simulink model "ZT_VehCtrl_18B_CAN"  (R2018b)
settings: Solver=FixedStepAuto  StartTime=0.0  StopTime=inf  FixedStep=0.005  RelTol=1e-3
InitFcn:
  | mbd_mpc_consistency_checks(bdroot(gcs));
values from neighbouring files (symbols this model uses):
  BatoverTempTh = single(80)    [VCU_INIT.m]
  BRS_PwrValid = single(5)    [VCU_INIT.m]
  BRSEnSpdTh1 = single(10)    [VCU_INIT.m]
  BRSEnSpdTh2 = single(20)    [VCU_INIT.m]
  MCUTempAlarmTh = single (60)    [VCU_INIT.m]
  mps2kmh = single(3.6)    [VCU_INIT.m]
  MtrPwrFac = single(1/9550)    [VCU_INIT.m]
  MtrTempAlarmTh = single (50)    [VCU_INIT.m]
  Padle1Signal1_Th = [PadleSignal1_min,PadleSignal1_max]    [VCU_INIT.m]
  Padle1Signal2_Th = [PadleSignal2_min,PadleSignal2_max]    [VCU_INIT.m]
  PadleSignal1_max = 3.84    [VCU_INIT.m]
  PadleSignal1_min = 0.75    [VCU_INIT.m]
  PadleSignal2_max = 1.92    [VCU_INIT.m]
  PadleSignal2_min = 0.375    [VCU_INIT.m]
  PadleValid = 0.05    [VCU_INIT.m]
  PwrLimFactor = single(0.5)    [VCU_INIT.m]
  Ratio = single(1)    [VCU_INIT.m]
  rpm2mps = single(2*pi/60 * WhlRadius/Ratio)    [VCU_INIT.m]
  SOCLowTh = single(20)    [VCU_INIT.m]
  VehPwrBackwardMax = VehPwrMax * single(0.3)    [VCU_INIT.m]
  VehPwrMax = single(MtrPwrMax * 4)    [VCU_INIT.m]
  VehTrqBackwardMax = VehTrqMax * single(0.3)    [VCU_INIT.m]
  VehTrqMax = single(MtrTrqMax * Ratio *4)    [VCU_INIT.m]
  WhlRadius = single(1)    [VCU_INIT.m]
undefined symbols (not defined in the file or in its folder): Delay_Charge, Delay_Discharge, fifo_0_vect, fifo_1_vect, LQFP, pts1_fifo_0_vect, pts1_fifo_1_vect, pts2_fifo_0_vect, pts2_fifo_1_vect, pts3_fifo_0_vect, pts3_fifo_1_vect, pts4_fifo_0_vect, pts4_fifo_1_vect
libraries: mbd_mpc574x_ec_toolbox x157, canmsglib x74, simulink x38
(part 7 of 12)

== system ZT_VehCtrl_18B_CAN/SigIn/CAN0 / BMS Power Control/UNPACK ==
  ID : Inport
  data : Inport  Port=2
  length : Inport  Port=3
  timestamp : Inport  Port=4
  Action Port : ActionPort
  Bus Creator : BusCreator  Inputs=7  OutDataTypeStr=Bus: CAN_MESSAGE_BUS  NonVirtualBus=on
  Bus Creator1 : BusCreator  Inputs=4
  CAN Unpack6 : canmsglib/CAN Unpack  CANdbFile=D:\VCU\VCU_SL_ZhengZhou\ZT2\模型与接口\CAN_DBC\整车CANA_GBK.dbc  MsgList=(none)  MsgName=BMS_Power_Control  MsgIDType=Standard (11-bit identifier)  MsgIdentifier=499  MsgLength=8  SignalInfo=Power_ChargeContinue$56$16$2$2$1$0$1.000000e-01$0$0$1000$#Power_ChargePeak$40$16$2$2$1$0$1.000000e-01$0$0$1000$#Power_DischargeContinue$24$16$2$2$1$0$1.000000e-01$0$0$1000$#Power_DischargePeak$8$16$2$2$1$0$1.000000e-01$0$0$1000$#  NSignals=4  IDPort=off  TimestampPort=off  ErrorPort=off  RemotePort=off  LengthPort=off  StatusPort=off  StartBits=str2num('[int32(56);int32(40);int32(24);int32(8)]')  SignalSizes=str2num('[int32(16);int32(16);int32(16);int32(16)]')  ByteOrders=str2num('[int32(2);int32(2);int32(2);int32(2)]')  DataTypes=str2num('[int32(2);int32(2);int32(2);int32(2)]')  MultiplexTypes=str2num('[int32(1);int32(1);int32(1);int32(1)]')  MultiplexValues=str2num('[double(0);double(0);double(0);double(0)]')  Factors=str2num('[double(1.000000e-01);double(1.000000e-01);double(1.000000e-01);double(1.000000e-01)]')  Offsets=str2num('[double(0);double(0);double(0);double(0)]')  Minimums=str2num('[double(0);double(0);double(0);double(0)]')  Maximums=str2num('[double(1000);double(1000);double(1000);double(1000)]')  ApplyMinMax=off
      settings: SourceProductName=Simulink Real-Time  SourceProductBaseCode=XP  DataFormat=CANdb specified signals
  Constant1 : Constant  Value=0  OutDataTypeStr=uint8
  Constant4 : Constant  Value=0  OutDataTypeStr=uint8
  Constant5 : Constant  Value=0  OutDataTypeStr=uint8
  Data Type Conversion{,14..15,17} (4 alike) : DataTypeConversion  OutDataTypeStr=uint8
  Data Type Conversion18 : DataTypeConversion  OutDataTypeStr=uint32
  Data Type Conversion19 : DataTypeConversion  OutDataTypeStr=double
  Message : Outport
  wires:
  Constant4/1 -> Data Type Conversion15/1
  length/1 -> Data Type Conversion14/1
  data/1 -> Bus Creator/7  "Data"
  Data Type Conversion18/1 -> Bus Creator/5  "ID"
  Constant1/1 -> Data Type Conversion/1
  Constant5/1 -> Data Type Conversion17/1
  ID/1 -> Data Type Conversion18/1
  Data Type Conversion19/1 -> Bus Creator/6  "Timestamp"
  timestamp/1 -> Data Type Conversion19/1
  Data Type Conversion17/1 -> Bus Creator/4  "Error"
  Bus Creator/1 -> CAN Unpack6/1  "CAN_Msg_In"
  Data Type Conversion/1 -> Bus Creator/1  "Extended"
  Data Type Conversion14/1 -> Bus Creator/2  "Length"
  Data Type Conversion15/1 -> Bus Creator/3  "Remote"
  Bus Creator1/1 -> Message/1

== system ZT_VehCtrl_18B_CAN/SigIn/CAN0 /ACU1/UNPACK ==
  ID : Inport
  data : Inport  Port=2
  length : Inport  Port=3
  timestamp : Inport  Port=4
  Action Port : ActionPort  ActionType=case
  Add : Sum
  Bus Creator : BusCreator  Inputs=7  OutDataTypeStr=Bus: CAN_MESSAGE_BUS  NonVirtualBus=on
  Bus Creator1 : BusCreator  Inputs=5
  CAN Unpack6 : canmsglib/CAN Unpack  CANdbFile=D:\VCU\VCU_SL_ZhengZhou\ZT2\模型与接口\CAN_DBC\动力CANB_GBK.dbc  MsgList=(none)  MsgName=ACU1  MsgIDType=Extended (29-bit identifier)  MsgIdentifier=201893786  MsgLength=8  SignalInfo=FaultCode$56$8$1$2$1$0$1$0$0$255$#InputVoltage$32$16$1$1$1$0$1.000000e-01$-1000$-1000$1000$#OutputCurrent$16$16$1$1$1$0$1.000000e-01$-1000$-1000$1000$#OutputVoltage$0$16$1$1$1$0$1.000000e-01$-1000$-1000$1000$#Temp$48$8$1$1$1$0$1$-50$-50$200$#  NSignals=5  IDPort=off  TimestampPort=off  ErrorPort=off  RemotePort=off  LengthPort=off  StatusPort=off  StartBits=str2num('[int32(56);int32(32);int32(16);int32(0);int32(48)]')  SignalSizes=str2num('[int32(8);int32(16);int32(16);int32(16);int32(8)]')  ByteOrders=str2num('[int32(1);int32(1);int32(1);int32(1);int32(1)]')  DataTypes=str2num('[int32(2);int32(1);int32(1);int32(1);int32(1)]')  MultiplexTypes=str2num('[int32(1);int32(1);int32(1);int32(1);int32(1)]')  MultiplexValues=str2num('[double(0);double(0);double(0);double(0);double(0)]')  Factors=str2num('[double(1);double(1.000000e-01);double(1.000000e-01);double(1.000000e-01);double(1)]')  Offsets=str2num('[double(0);double(-1000);double(-1000);double(-1000);double(-50)]')  Minimums=str2num('[double(0);double(-1000);double(-1000);double(-1000);double(-50)]')  Maximums=str2num('[double(255);double(1000);double(1000);double(1000);double(200)]')  ApplyMinMax=off
      settings: SourceProductName=Simulink Real-Time  SourceProductBaseCode=XP  DataFormat=CANdb specified signals
  Constant : Constant  OutDataTypeStr=uint8
  Constant1 : Constant  OutDataTypeStr=uint8
  Constant4 : Constant  Value=0  OutDataTypeStr=uint8
  Constant5 : Constant  Value=0  OutDataTypeStr=uint8
  Data Store Read : DataStoreRead  DataStoreName=Cnt_ACU1
  Data Store Write : DataStoreWrite  DataStoreName=Cnt_ACU1
  Data Type Conversion{,14..15,17} (4 alike) : DataTypeConversion  OutDataTypeStr=uint8
  Data Type Conversion{1..5} (5 alike) : DataTypeConversion  OutDataTypeStr=single
  Data Type Conversion18 : DataTypeConversion  OutDataTypeStr=uint32
  Data Type Conversion19 : DataTypeConversion  OutDataTypeStr=double
  Message : Outport
  wires:
  Constant4/1 -> Data Type Conversion15/1
  length/1 -> Data Type Conversion14/1
  data/1 -> Bus Creator/7  "Data"
  Data Type Conversion18/1 -> Bus Creator/5  "ID"
  Constant1/1 -> Data Type Conversion/1
  Constant5/1 -> Data Type Conversion17/1
  ID/1 -> Data Type Conversion18/1
  Data Type Conversion19/1 -> Bus Creator/6  "Timestamp"
  timestamp/1 -> Data Type Conversion19/1
  Data Type Conversion17/1 -> Bus Creator/4  "Error"
  Bus Creator/1 -> CAN Unpack6/1  "CAN_Msg_In"
  Data Type Conversion/1 -> Bus Creator/1  "Extended"
  Data Type Conversion14/1 -> Bus Creator/2  "Length"
  Data Type Conversion15/1 -> Bus Creator/3  "Remote"
  Bus Creator1/1 -> Message/1
  CAN Unpack6/1 -> Data Type Conversion1/1
  CAN Unpack6/2 -> Data Type Conversion2/1
  CAN Unpack6/3 -> Data Type Conversion3/1
  CAN Unpack6/4 -> Data Type Conversion4/1
  CAN Unpack6/5 -> Data Type Conversion5/1
  Data Type Conversion1/1 -> Bus Creator1/1  "FaultCode"
  Data Type Conversion2/1 -> Bus Creator1/2  "InputVoltage"
  Data Type Conversion3/1 -> Bus Creator1/3  "OutputCurrent"
  Data Type Conversion4/1 -> Bus Creator1/4  "OutputVoltage"
  Data Type Conversion5/1 -> Bus Creator1/5  "Temp"
  Constant/1 -> Add/2
  Data Store Read/1 -> Add/1
  Add/1 -> Data Store Write/1

== system ZT_VehCtrl_18B_CAN/SigIn/CAN0 /ACU2/UNPACK ==
  ID : Inport
  data : Inport  Port=2
  length : Inport  Port=3
  timestamp : Inport  Port=4
  Action Port : ActionPort  ActionType=case
  Add : Sum
  Bus Creator : BusCreator  Inputs=7  OutDataTypeStr=Bus: CAN_MESSAGE_BUS  NonVirtualBus=on
  Bus Creator1 : BusCreator  Inputs=5
  CAN Unpack6 : canmsglib/CAN Unpack  CANdbFile=D:\VCU\VCU_SL_ZhengZhou\ZT2\模型与接口\CAN_DBC\动力CANB_GBK.dbc  MsgList=(none)  MsgName=ACU2  MsgIDType=Extended (29-bit identifier)  MsgIdentifier=201959323  MsgLength=8  SignalInfo=CurrentU$32$16$1$1$1$0$1.000000e-01$-1000$-1000$1000$#CurrentV$16$16$1$1$1$0$1.000000e-01$-1000$-1000$1000$#CurrentW$0$16$1$1$1$0$1.000000e-01$-1000$-1000$1000$#FaultCode$56$8$1$2$1$0$1$0$0$255$#Temp$48$8$1$1$1$0$1$-50$-50$200$#  NSignals=5  IDPort=off  TimestampPort=off  ErrorPort=off  RemotePort=off  LengthPort=off  StatusPort=off  StartBits=str2num('[int32(32);int32(16);int32(0);int32(56);int32(48)]')  SignalSizes=str2num('[int32(16);int32(16);int32(16);int32(8);int32(8)]')  ByteOrders=str2num('[int32(1);int32(1);int32(1);int32(1);int32(1)]')  DataTypes=str2num('[int32(1);int32(1);int32(1);int32(2);int32(1)]')  MultiplexTypes=str2num('[int32(1);int32(1);int32(1);int32(1);int32(1)]')  MultiplexValues=str2num('[double(0);double(0);double(0);double(0);double(0)]')  Factors=str2num('[double(1.000000e-01);double(1.000000e-01);double(1.000000e-01);double(1);double(1)]')  Offsets=str2num('[double(-1000);double(-1000);double(-1000);double(0);double(-50)]')  Minimums=str2num('[double(-1000);double(-1000);double(-1000);double(0);double(-50)]')  Maximums=str2num('[double(1000);double(1000);double(1000);double(255);double(200)]')  ApplyMinMax=off
      settings: SourceProductName=Simulink Real-Time  SourceProductBaseCode=XP  DataFormat=CANdb specified signals
  Constant : Constant  OutDataTypeStr=uint8
  Constant1 : Constant  OutDataTypeStr=uint8
  Constant4 : Constant  Value=0  OutDataTypeStr=uint8
  Constant5 : Constant  Value=0  OutDataTypeStr=uint8
  Data Store Read : DataStoreRead  DataStoreName=Cnt_ACU2
  Data Store Write : DataStoreWrite  DataStoreName=Cnt_ACU2
  Data Type Conversion{,14..15,17} (4 alike) : DataTypeConversion  OutDataTypeStr=uint8
  Data Type Conversion{1..5} (5 alike) : DataTypeConversion  OutDataTypeStr=single
  Data Type Conversion18 : DataTypeConversion  OutDataTypeStr=uint32
  Data Type Conversion19 : DataTypeConversion  OutDataTypeStr=double
  Message : Outport
  wires:
  Bus Creator1/1 -> Message/1
  Data Type Conversion15/1 -> Bus Creator/3  "Remote"
  Data Type Conversion14/1 -> Bus Creator/2  "Length"
  Data Type Conversion/1 -> Bus Creator/1  "Extended"
  Bus Creator/1 -> CAN Unpack6/1  "CAN_Msg_In"
  Data Type Conversion17/1 -> Bus Creator/4  "Error"
  timestamp/1 -> Data Type Conversion19/1
  Data Type Conversion19/1 -> Bus Creator/6  "Timestamp"
  ID/1 -> Data Type Conversion18/1
  Constant5/1 -> Data Type Conversion17/1
  Constant1/1 -> Data Type Conversion/1
  Data Type Conversion18/1 -> Bus Creator/5  "ID"
  data/1 -> Bus Creator/7  "Data"
  length/1 -> Data Type Conversion14/1
  Constant4/1 -> Data Type Conversion15/1
  CAN Unpack6/1 -> Data Type Conversion1/1
  CAN Unpack6/2 -> Data Type Conversion2/1
  CAN Unpack6/3 -> Data Type Conversion3/1
  CAN Unpack6/4 -> Data Type Conversion4/1
  CAN Unpack6/5 -> Data Type Conversion5/1
  Data Type Conversion1/1 -> Bus Creator1/1  "CurrentU"
  Data Type Conversion2/1 -> Bus Creator1/2  "CurrentV"
  Data Type Conversion3/1 -> Bus Creator1/3  "CurrentW"
  Data Type Conversion4/1 -> Bus Creator1/4  "FaultCode"
  Data Type Conversion5/1 -> Bus Creator1/5  "Temp"
  Add/1 -> Data Store Write/1
  Data Store Read/1 -> Add/1
  Constant/1 -> Add/2

== system ZT_VehCtrl_18B_CAN/SigIn/CAN0 /ACU3/UNPACK ==
  ID : Inport
  data : Inport  Port=2
  length : Inport  Port=3
  timestamp : Inport  Port=4
  Action Port : ActionPort  ActionType=case
  Add : Sum
  Bus Creator : BusCreator  Inputs=7  OutDataTypeStr=Bus: CAN_MESSAGE_BUS  NonVirtualBus=on
  Bus Creator1 : BusCreator  Inputs=5
  CAN Unpack6 : canmsglib/CAN Unpack  CANdbFile=D:\VCU\VCU_SL_ZhengZhou\ZT2\模型与接口\CAN_DBC\动力CANB_GBK.dbc  MsgList=(none)  MsgName=ACU3  MsgIDType=Extended (29-bit identifier)  MsgIdentifier=202024861  MsgLength=8  SignalInfo=CurrentU$32$16$1$1$1$0$1.000000e-01$-1000$-1000$1000$#CurrentV$16$16$1$1$1$0$1.000000e-01$-1000$-1000$1000$#CurrentW$0$16$1$1$1$0$1.000000e-01$-1000$-1000$1000$#FaultCode$56$8$1$2$1$0$1$0$0$255$#Temp$48$8$1$1$1$0$1$-50$-50$200$#  NSignals=5  IDPort=off  TimestampPort=off  ErrorPort=off  RemotePort=off  LengthPort=off  StatusPort=off  StartBits=str2num('[int32(32);int32(16);int32(0);int32(56);int32(48)]')  SignalSizes=str2num('[int32(16);int32(16);int32(16);int32(8);int32(8)]')  ByteOrders=str2num('[int32(1);int32(1);int32(1);int32(1);int32(1)]')  DataTypes=str2num('[int32(1);int32(1);int32(1);int32(2);int32(1)]')  MultiplexTypes=str2num('[int32(1);int32(1);int32(1);int32(1);int32(1)]')  MultiplexValues=str2num('[double(0);double(0);double(0);double(0);double(0)]')  Factors=str2num('[double(1.000000e-01);double(1.000000e-01);double(1.000000e-01);double(1);double(1)]')  Offsets=str2num('[double(-1000);double(-1000);double(-1000);double(0);double(-50)]')  Minimums=str2num('[double(-1000);double(-1000);double(-1000);double(0);double(-50)]')  Maximums=str2num('[double(1000);double(1000);double(1000);double(255);double(200)]')  ApplyMinMax=off
      settings: SourceProductName=Simulink Real-Time  SourceProductBaseCode=XP  DataFormat=CANdb specified signals
  Constant : Constant  OutDataTypeStr=uint8
  Constant1 : Constant  OutDataTypeStr=uint8
  Constant4 : Constant  Value=0  OutDataTypeStr=uint8
  Constant5 : Constant  Value=0  OutDataTypeStr=uint8
  Data Store Read : DataStoreRead  DataStoreName=Cnt_ACU3
  Data Store Write : DataStoreWrite  DataStoreName=Cnt_ACU3
  Data Type Conversion{,14..15,17} (4 alike) : DataTypeConversion  OutDataTypeStr=uint8
  Data Type Conversion{1..5} (5 alike) : DataTypeConversion  OutDataTypeStr=single
  Data Type Conversion18 : DataTypeConversion  OutDataTypeStr=uint32
  Data Type Conversion19 : DataTypeConversion  OutDataTypeStr=double
  Message : Outport
  wires:
  Constant4/1 -> Data Type Conversion15/1
  length/1 -> Data Type Conversion14/1
  data/1 -> Bus Creator/7  "Data"
  Data Type Conversion18/1 -> Bus Creator/5  "ID"
  Constant1/1 -> Data Type Conversion/1
  Constant5/1 -> Data Type Conversion17/1
  ID/1 -> Data Type Conversion18/1
  Data Type Conversion19/1 -> Bus Creator/6  "Timestamp"
  timestamp/1 -> Data Type Conversion19/1
  Data Type Conversion17/1 -> Bus Creator/4  "Error"
  Bus Creator/1 -> CAN Unpack6/1  "CAN_Msg_In"
  Data Type Conversion/1 -> Bus Creator/1  "Extended"
  Data Type Conversion14/1 -> Bus Creator/2  "Length"
  Data Type Conversion15/1 -> Bus Creator/3  "Remote"
  Data Type Conversion5/1 -> Bus Creator1/5  "Temp"
  Data Type Conversion3/1 -> Bus Creator1/3  "CurrentW"
  Data Type Conversion2/1 -> Bus Creator1/2  "CurrentV"
  Data Type Conversion1/1 -> Bus Creator1/1  "CurrentU"
  Data Type Conversion4/1 -> Bus Creator1/4  "FaultCode"
  Bus Creator1/1 -> Message/1
  CAN Unpack6/1 -> Data Type Conversion1/1
  CAN Unpack6/2 -> Data Type Conversion2/1
  CAN Unpack6/3 -> Data Type Conversion3/1
  CAN Unpack6/4 -> Data Type Conversion4/1
  CAN Unpack6/5 -> Data Type Conversion5/1
  Add/1 -> Data Store Write/1
  Data Store Read/1 -> Add/1
  Constant/1 -> Add/2

== system ZT_VehCtrl_18B_CAN/SigIn/CAN0 /BMS Cell Battery Temperature/UNPACK ==
  ID : Inport
  data : Inport  Port=2
  length : Inport  Port=3
  timestamp : Inport  Port=4
  Action Port : ActionPort
  Bus Creator : BusCreator  Inputs=7  OutDataTypeStr=Bus: CAN_MESSAGE_BUS  NonVirtualBus=on
  Bus Creator1 : BusCreator  Inputs=2
  CAN Unpack6 : canmsglib/CAN Unpack  CANdbFile=D:\VCU\VCU_SL_ZhengZhou\ZT2\模型与接口\CAN_DBC\整车CANA_GBK.dbc  MsgList=(none)  MsgName=BMS_Cell_Battery_Temperature  MsgIDType=Standard (11-bit identifier)  MsgIdentifier=855  MsgLength=8  SignalInfo=CellTempearture_T1$16$8$2$2$1$0$1$-50$-50$125$#CellTempearture_T2$24$8$2$2$1$0$1$-50$-50$125$#CellTempearture_T3$32$8$2$2$1$0$1$-50$-50$125$#CellTempearture_T4$40$8$2$2$1$0$1$-50$-50$125$#CellTempearture_T5$48$8$2$2$1$0$1$-50$-50$125$#CellTempearture_T6$56$8$2$2$1$0$1$-50$-50$125$#CellTemperature_StartNum$8$16$2$2$1$0$1$0$0$1000$#  NSignals=7  IDPort=off  TimestampPort=off  ErrorPort=off  RemotePort=off  LengthPort=off  StatusPort=off  StartBits=str2num('[int32(16);int32(24);int32(32);int32(40);int32(48);int32(56);int32(8)]')  SignalSizes=str2num('[int32(8);int32(8);int32(8);int32(8);int32(8);int32(8);int32(16)]')  ByteOrders=str2num('[int32(2);int32(2);int32(2);int32(2);int32(2);int32(2);int32(2)]')  DataTypes=str2num('[int32(2);int32(2);int32(2);int32(2);int32(2);int32(2);int32(2)]')  MultiplexTypes=str2num('[int32(1);int32(1);int32(1);int32(1);int32(1);int32(1);int32(1)]')  MultiplexValues=str2num('[double(0);double(0);double(0);double(0);double(0);double(0);double(0)]')  Factors=str2num('[double(1);double(1);double(1);double(1);double(1);double(1);double(1)]')  Offsets=str2num('[double(-50);double(-50);double(-50);double(-50);double(-50);double(-50);double(0)]')  Minimums=str2num('[double(-50);double(-50);double(-50);double(-50);double(-50);double(-50);double(0)]')  Maximums=str2num('[double(125);double(125);double(125);double(125);double(125);double(125);double(1000)]')  ApplyMinMax=off
      settings: SourceProductName=Simulink Real-Time  SourceProductBaseCode=XP  DataFormat=CANdb specified signals
  Constant1 : Constant  Value=0  OutDataTypeStr=uint8
  Constant4 : Constant  Value=0  OutDataTypeStr=uint8
  Constant5 : Constant  Value=0  OutDataTypeStr=uint8
  Data Type Conversion{,14..15,17} (4 alike) : DataTypeConversion  OutDataTypeStr=uint8
  Data Type Conversion18 : DataTypeConversion  OutDataTypeStr=uint32
  Data Type Conversion19 : DataTypeConversion  OutDataTypeStr=double
  Message : Outport
  wires:
  Bus Creator1/1 -> Message/1
  Data Type Conversion15/1 -> Bus Creator/3  "Remote"
  Data Type Conversion14/1 -> Bus Creator/2  "Length"
  Data Type Conversion/1 -> Bus Creator/1  "Extended"
  Bus Creator/1 -> CAN Unpack6/1  "CAN_Msg_In"
  Data Type Conversion17/1 -> Bus Creator/4  "Error"
  timestamp/1 -> Data Type Conversion19/1
  Data Type Conversion19/1 -> Bus Creator/6  "Timestamp"
  ID/1 -> Data Type Conversion18/1
  Constant5/1 -> Data Type Conversion17/1
  Constant1/1 -> Data Type Conversion/1
  Data Type Conversion18/1 -> Bus Creator/5  "ID"
  data/1 -> Bus Creator/7  "Data"
  length/1 -> Data Type Conversion14/1
  Constant4/1 -> Data Type Conversion15/1

== system ZT_VehCtrl_18B_CAN/SigIn/CAN0 /BMS Cell HeatingTemperature/UNPACK ==
  ID : Inport
  data : Inport  Port=2
  length : Inport  Port=3
  timestamp : Inport  Port=4
  Action Port : ActionPort
  Bus Creator : BusCreator  Inputs=7  OutDataTypeStr=Bus: CAN_MESSAGE_BUS  NonVirtualBus=on
  Bus Creator1 : BusCreator  Inputs=2
  CAN Unpack6 : canmsglib/CAN Unpack  CANdbFile=D:\VCU\VCU_SL_ZhengZhou\ZT2\模型与接口\CAN_DBC\整车CANA_GBK.dbc  MsgList=(none)  MsgName=BMS_Cell_HeatingTemperature  MsgIDType=Standard (11-bit identifier)  MsgIdentifier=1011  MsgLength=8  SignalInfo=CellHeatingTempearture_T1$16$8$2$2$1$0$1$-50$-50$125$#CellHeatingTempearture_T2$24$8$2$2$1$0$1$-50$-50$125$#CellHeatingTempearture_T3$32$8$2$2$1$0$1$-50$-50$125$#CellHeatingTempearture_T4$40$8$2$2$1$0$1$-50$-50$125$#CellHeatingTempearture_T5$48$8$2$2$1$0$1$-50$-50$125$#CellHeatingTempearture_T6$56$8$2$2$1$0$1$-50$-50$125$#CellHeatingTemperature_StartNum$8$16$2$2$1$0$1$0$0$1000$#  NSignals=7  IDPort=off  TimestampPort=off  ErrorPort=off  RemotePort=off  LengthPort=off  StatusPort=off  StartBits=str2num('[int32(16);int32(24);int32(32);int32(40);int32(48);int32(56);int32(8)]')  SignalSizes=str2num('[int32(8);int32(8);int32(8);int32(8);int32(8);int32(8);int32(16)]')  ByteOrders=str2num('[int32(2);int32(2);int32(2);int32(2);int32(2);int32(2);int32(2)]')  DataTypes=str2num('[int32(2);int32(2);int32(2);int32(2);int32(2);int32(2);int32(2)]')  MultiplexTypes=str2num('[int32(1);int32(1);int32(1);int32(1);int32(1);int32(1);int32(1)]')  MultiplexValues=str2num('[double(0);double(0);double(0);double(0);double(0);double(0);double(0)]')  Factors=str2num('[double(1);double(1);double(1);double(1);double(1);double(1);double(1)]')  Offsets=str2num('[double(-50);double(-50);double(-50);double(-50);double(-50);double(-50);double(0)]')  Minimums=str2num('[double(-50);double(-50);double(-50);double(-50);double(-50);double(-50);double(0)]')  Maximums=str2num('[double(125);double(125);double(125);double(125);double(125);double(125);double(1000)]')  ApplyMinMax=off
      settings: SourceProductName=Simulink Real-Time  SourceProductBaseCode=XP  DataFormat=CANdb specified signals
  Constant1 : Constant  Value=0  OutDataTypeStr=uint8
  Constant4 : Constant  Value=0  OutDataTypeStr=uint8
  Constant5 : Constant  Value=0  OutDataTypeStr=uint8
  Data Type Conversion{,14..15,17} (4 alike) : DataTypeConversion  OutDataTypeStr=uint8
  Data Type Conversion18 : DataTypeConversion  OutDataTypeStr=uint32
  Data Type Conversion19 : DataTypeConversion  OutDataTypeStr=double
  Message : Outport
  wires:
  Constant4/1 -> Data Type Conversion15/1
  length/1 -> Data Type Conversion14/1
  data/1 -> Bus Creator/7  "Data"
  Data Type Conversion18/1 -> Bus Creator/5  "ID"
  Constant1/1 -> Data Type Conversion/1
  Constant5/1 -> Data Type Conversion17/1
  ID/1 -> Data Type Conversion18/1
  Data Type Conversion19/1 -> Bus Creator/6  "Timestamp"
  timestamp/1 -> Data Type Conversion19/1
  Data Type Conversion17/1 -> Bus Creator/4  "Error"
  Bus Creator/1 -> CAN Unpack6/1  "CAN_Msg_In"
  Data Type Conversion/1 -> Bus Creator/1  "Extended"
  Data Type Conversion14/1 -> Bus Creator/2  "Length"
  Data Type Conversion15/1 -> Bus Creator/3  "Remote"
  Bus Creator1/1 -> Message/1

== system ZT_VehCtrl_18B_CAN/SigIn/CAN0 /BMS Cell Pole Temperature/UNPACK ==
  ID : Inport
  data : Inport  Port=2
  length : Inport  Port=3
  timestamp : Inport  Port=4
  Action Port : ActionPort
  Bus Creator : BusCreator  Inputs=7  OutDataTypeStr=Bus: CAN_MESSAGE_BUS  NonVirtualBus=on
  Bus Creator1 : BusCreator  Inputs=2
  CAN Unpack6 : canmsglib/CAN Unpack  CANdbFile=D:\VCU\VCU_SL_ZhengZhou\ZT2\模型与接口\CAN_DBC\整车CANA_GBK.dbc  MsgList=(none)  MsgName=BMS_Cell_Pole_Temperature  MsgIDType=Standard (11-bit identifier)  MsgIdentifier=1012  MsgLength=8  SignalInfo=CellPoleTempearture_T1$16$8$2$2$1$0$1$-50$-50$125$#CellPoleTempearture_T2$24$8$2$2$1$0$1$-50$-50$125$#CellPoleTempearture_T3$32$8$2$2$1$0$1$-50$-50$125$#CellPoleTempearture_T4$40$8$2$2$1$0$1$-50$-50$125$#CellPoleTempearture_T5$48$8$2$2$1$0$1$-50$-50$125$#CellPoleTempearture_T6$56$8$2$2$1$0$1$-50$-50$125$#CellPoleTemperature_StartNum$8$16$2$2$1$0$1$0$0$1000$#  NSignals=7  IDPort=off  TimestampPort=off  ErrorPort=off  RemotePort=off  LengthPort=off  StatusPort=off  StartBits=str2num('[int32(16);int32(24);int32(32);int32(40);int32(48);int32(56);int32(8)]')  SignalSizes=str2num('[int32(8);int32(8);int32(8);int32(8);int32(8);int32(8);int32(16)]')  ByteOrders=str2num('[int32(2);int32(2);int32(2);int32(2);int32(2);int32(2);int32(2)]')  DataTypes=str2num('[int32(2);int32(2);int32(2);int32(2);int32(2);int32(2);int32(2)]')  MultiplexTypes=str2num('[int32(1);int32(1);int32(1);int32(1);int32(1);int32(1);int32(1)]')  MultiplexValues=str2num('[double(0);double(0);double(0);double(0);double(0);double(0);double(0)]')  Factors=str2num('[double(1);double(1);double(1);double(1);double(1);double(1);double(1)]')  Offsets=str2num('[double(-50);double(-50);double(-50);double(-50);double(-50);double(-50);double(0)]')  Minimums=str2num('[double(-50);double(-50);double(-50);double(-50);double(-50);double(-50);double(0)]')  Maximums=str2num('[double(125);double(125);double(125);double(125);double(125);double(125);double(1000)]')  ApplyMinMax=off
      settings: SourceProductName=Simulink Real-Time  SourceProductBaseCode=XP  DataFormat=CANdb specified signals
  Constant1 : Constant  Value=0  OutDataTypeStr=uint8
  Constant4 : Constant  Value=0  OutDataTypeStr=uint8
  Constant5 : Constant  Value=0  OutDataTypeStr=uint8
  Data Type Conversion{,14..15,17} (4 alike) : DataTypeConversion  OutDataTypeStr=uint8
  Data Type Conversion18 : DataTypeConversion  OutDataTypeStr=uint32
  Data Type Conversion19 : DataTypeConversion  OutDataTypeStr=double
  Message : Outport
  wires:
  Bus Creator1/1 -> Message/1
  Data Type Conversion15/1 -> Bus Creator/3  "Remote"
  Data Type Conversion14/1 -> Bus Creator/2  "Length"
  Data Type Conversion/1 -> Bus Creator/1  "Extended"
  Bus Creator/1 -> CAN Unpack6/1  "CAN_Msg_In"
  Data Type Conversion17/1 -> Bus Creator/4  "Error"
  timestamp/1 -> Data Type Conversion19/1
  Data Type Conversion19/1 -> Bus Creator/6  "Timestamp"
  ID/1 -> Data Type Conversion18/1
  Constant5/1 -> Data Type Conversion17/1
  Constant1/1 -> Data Type Conversion/1
  Data Type Conversion18/1 -> Bus Creator/5  "ID"
  data/1 -> Bus Creator/7  "Data"
  length/1 -> Data Type Conversion14/1
  Constant4/1 -> Data Type Conversion15/1

== system ZT_VehCtrl_18B_CAN/SigIn/CAN0 /BMS Cell Voltage Infor/UNPACK ==
  ID : Inport
  data : Inport  Port=2
  length : Inport  Port=3
  timestamp : Inport  Port=4
  Action Port : ActionPort
  Bus Creator : BusCreator  Inputs=7  OutDataTypeStr=Bus: CAN_MESSAGE_BUS  NonVirtualBus=on
  Bus Creator1 : BusCreator  Inputs=4
  CAN Unpack6 : canmsglib/CAN Unpack  CANdbFile=D:\VCU\VCU_SL_ZhengZhou\ZT2\模型与接口\CAN_DBC\整车CANA_GBK.dbc  MsgList=(none)  MsgName=BMS_Cell_Voltage_Infor  MsgIDType=Standard (11-bit identifier)  MsgIdentifier=854  MsgLength=8  SignalInfo=CellVoltage_StartNum$8$16$2$2$1$0$1$0$0$1000$#CellVoltage_V1$24$16$2$2$1$0$1.000000e-03$0$0$10$#CellVoltage_V2$40$16$2$2$1$0$1.000000e-03$0$0$10$#CellVoltage_V3$56$16$2$2$1$0$1.000000e-03$0$0$10$#  NSignals=4  IDPort=off  TimestampPort=off  ErrorPort=off  RemotePort=off  LengthPort=off  StatusPort=off  StartBits=str2num('[int32(8);int32(24);int32(40);int32(56)]')  SignalSizes=str2num('[int32(16);int32(16);int32(16);int32(16)]')  ByteOrders=str2num('[int32(2);int32(2);int32(2);int32(2)]')  DataTypes=str2num('[int32(2);int32(2);int32(2);int32(2)]')  MultiplexTypes=str2num('[int32(1);int32(1);int32(1);int32(1)]')  MultiplexValues=str2num('[double(0);double(0);double(0);double(0)]')  Factors=str2num('[double(1);double(1.000000e-03);double(1.000000e-03);double(1.000000e-03)]')  Offsets=str2num('[double(0);double(0);double(0);double(0)]')  Minimums=str2num('[double(0);double(0);double(0);double(0)]')  Maximums=str2num('[double(1000);double(10);double(10);double(10)]')  ApplyMinMax=off
      settings: SourceProductName=Simulink Real-Time  SourceProductBaseCode=XP  DataFormat=CANdb specified signals
  Constant1 : Constant  Value=0  OutDataTypeStr=uint8
  Constant4 : Constant  Value=0  OutDataTypeStr=uint8
  Constant5 : Constant  Value=0  OutDataTypeStr=uint8
  Data Type Conversion{,14..15,17} (4 alike) : DataTypeConversion  OutDataTypeStr=uint8
  Data Type Conversion18 : DataTypeConversion  OutDataTypeStr=uint32
  Data Type Conversion19 : DataTypeConversion  OutDataTypeStr=double
  Message : Outport
  wires:
  Bus Creator1/1 -> Message/1
  Data Type Conversion15/1 -> Bus Creator/3  "Remote"
  Data Type Conversion14/1 -> Bus Creator/2  "Length"
  Data Type Conversion/1 -> Bus Creator/1  "Extended"
  Bus Creator/1 -> CAN Unpack6/1  "CAN_Msg_In"
  Data Type Conversion17/1 -> Bus Creator/4  "Error"
  timestamp/1 -> Data Type Conversion19/1
  Data Type Conversion19/1 -> Bus Creator/6  "Timestamp"
  ID/1 -> Data Type Conversion18/1
  Constant5/1 -> Data Type Conversion17/1
  Constant1/1 -> Data Type Conversion/1
  Data Type Conversion18/1 -> Bus Creator/5  "ID"
  data/1 -> Bus Creator/7  "Data"
  length/1 -> Data Type Conversion14/1
  Constant4/1 -> Data Type Conversion15/1

== system ZT_VehCtrl_18B_CAN/SigIn/CAN0 /BMS CumuCap Infor/UNPACK ==
  ID : Inport
  data : Inport  Port=2
  length : Inport  Port=3
  timestamp : Inport  Port=4
  Action Port : ActionPort
  Bus Creator : BusCreator  Inputs=7  OutDataTypeStr=Bus: CAN_MESSAGE_BUS  NonVirtualBus=on
  Bus Creator1 : BusCreator  Inputs=2
  CAN Unpack6 : canmsglib/CAN Unpack  CANdbFile=D:\VCU\VCU_SL_ZhengZhou\ZT2\模型与接口\CAN_DBC\整车CANA_GBK.dbc  MsgList=(none)  MsgName=BMS_CumuCap_Infor  MsgIDType=Standard (11-bit identifier)  MsgIdentifier=1013  MsgLength=8  SignalInfo=CumuCap_Charge$56$32$2$2$1$0$1$0$0$4294967295$#CumuCap_Discharge$24$32$2$2$1$0$1$0$0$4294967295$#  NSignals=2  IDPort=off  TimestampPort=off  ErrorPort=off  RemotePort=off  LengthPort=off  StatusPort=off  StartBits=str2num('[int32(56);int32(24)]')  SignalSizes=str2num('[int32(32);int32(32)]')  ByteOrders=str2num('[int32(2);int32(2)]')  DataTypes=str2num('[int32(2);int32(2)]')  MultiplexTypes=str2num('[int32(1);int32(1)]')  MultiplexValues=str2num('[double(0);double(0)]')  Factors=str2num('[double(1);double(1)]')  Offsets=str2num('[double(0);double(0)]')  Minimums=str2num('[double(0);double(0)]')  Maximums=str2num('[double(4294967295);double(4294967295)]')  ApplyMinMax=off
      settings: SourceProductName=Simulink Real-Time  SourceProductBaseCode=XP  DataFormat=CANdb specified signals
  Constant1 : Constant  Value=0  OutDataTypeStr=uint8
  Constant4 : Constant  Value=0  OutDataTypeStr=uint8
  Constant5 : Constant  Value=0  OutDataTypeStr=uint8
  Data Type Conversion{,14..15,17} (4 alike) : DataTypeConversion  OutDataTypeStr=uint8
  Data Type Conversion18 : DataTypeConversion  OutDataTypeStr=uint32
  Data Type Conversion19 : DataTypeConversion  OutDataTypeStr=double
  Message : Outport
  wires:
  Constant4/1 -> Data Type Conversion15/1
  length/1 -> Data Type Conversion14/1
  data/1 -> Bus Creator/7  "Data"
  Data Type Conversion18/1 -> Bus Creator/5  "ID"
  Constant1/1 -> Data Type Conversion/1
  Constant5/1 -> Data Type Conversion17/1
  ID/1 -> Data Type Conversion18/1
  Data Type Conversion19/1 -> Bus Creator/6  "Timestamp"
  timestamp/1 -> Data Type Conversion19/1
  Data Type Conversion17/1 -> Bus Creator/4  "Error"
  Bus Creator/1 -> CAN Unpack6/1  "CAN_Msg_In"
  Data Type Conversion/1 -> Bus Creator/1  "Extended"
  Data Type Conversion14/1 -> Bus Creator/2  "Length"
  Data Type Conversion15/1 -> Bus Creator/3  "Remote"
  Bus Creator1/1 -> Message/1

== system ZT_VehCtrl_18B_CAN/SigIn/CAN0 /BMS CumuTimeInfor1/UNPACK ==
  ID : Inport
  data : Inport  Port=2
  length : Inport  Port=3
  timestamp : Inport  Port=4
  Action Port : ActionPort
  Bus Creator : BusCreator  Inputs=7  OutDataTypeStr=Bus: CAN_MESSAGE_BUS  NonVirtualBus=on
  Bus Creator1 : BusCreator  Inputs=2
  CAN Unpack6 : canmsglib/CAN Unpack  CANdbFile=D:\VCU\VCU_SL_ZhengZhou\ZT2\模型与接口\CAN_DBC\整车CANA_GBK.dbc  MsgList=(none)  MsgName=BMS_CumuTimeInfor1  MsgIDType=Standard (11-bit identifier)  MsgIdentifier=515  MsgLength=8  SignalInfo=CumuTime_Charge$56$32$2$2$1$0$1.000000e-01$0$0$4294967295$#CumuTime_Discharge$24$32$2$2$1$0$1.000000e-01$0$0$4294967295$#  NSignals=2  IDPort=off  TimestampPort=off  ErrorPort=off  RemotePort=off  LengthPort=off  StatusPort=off  StartBits=str2num('[int32(56);int32(24)]')  SignalSizes=str2num('[int32(32);int32(32)]')  ByteOrders=str2num('[int32(2);int32(2)]')  DataTypes=str2num('[int32(2);int32(2)]')  MultiplexTypes=str2num('[int32(1);int32(1)]')  MultiplexValues=str2num('[double(0);double(0)]')  Factors=str2num('[double(1.000000e-01);double(1.000000e-01)]')  Offsets=str2num('[double(0);double(0)]')  Minimums=str2num('[double(0);double(0)]')  Maximums=str2num('[double(4294967295);double(4294967295)]')  ApplyMinMax=off
      settings: SourceProductName=Simulink Real-Time  SourceProductBaseCode=XP  DataFormat=CANdb specified signals
  Constant1 : Constant  Value=0  OutDataTypeStr=uint8
  Constant4 : Constant  Value=0  OutDataTypeStr=uint8
  Constant5 : Constant  Value=0  OutDataTypeStr=uint8
  Data Type Conversion{,14..15,17} (4 alike) : DataTypeConversion  OutDataTypeStr=uint8
  Data Type Conversion18 : DataTypeConversion  OutDataTypeStr=uint32
  Data Type Conversion19 : DataTypeConversion  OutDataTypeStr=double
  Message : Outport
  wires:
  Bus Creator1/1 -> Message/1
  Data Type Conversion15/1 -> Bus Creator/3  "Remote"
  Data Type Conversion14/1 -> Bus Creator/2  "Length"
  Data Type Conversion/1 -> Bus Creator/1  "Extended"
  Bus Creator/1 -> CAN Unpack6/1  "CAN_Msg_In"
  Data Type Conversion17/1 -> Bus Creator/4  "Error"
  timestamp/1 -> Data Type Conversion19/1
  Data Type Conversion19/1 -> Bus Creator/6  "Timestamp"
  ID/1 -> Data Type Conversion18/1
  Constant5/1 -> Data Type Conversion17/1
  Constant1/1 -> Data Type Conversion/1
  Data Type Conversion18/1 -> Bus Creator/5  "ID"
  data/1 -> Bus Creator/7  "Data"
  length/1 -> Data Type Conversion14/1
  Constant4/1 -> Data Type Conversion15/1

== system ZT_VehCtrl_18B_CAN/SigIn/CAN0 /BMS CumuTimeInfor2/UNPACK ==
  ID : Inport
  data : Inport  Port=2
  length : Inport  Port=3
  timestamp : Inport  Port=4
  Action Port : ActionPort
  Bus Creator : BusCreator  Inputs=7  OutDataTypeStr=Bus: CAN_MESSAGE_BUS  NonVirtualBus=on
  Bus Creator1 : BusCreator  Inputs=2
  CAN Unpack6 : canmsglib/CAN Unpack  CANdbFile=D:\VCU\VCU_SL_ZhengZhou\ZT2\模型与接口\CAN_DBC\整车CANA_GBK.dbc  MsgList=(none)  MsgName=BMS_CumuTimeInfor2  MsgIDType=Standard (11-bit identifier)  MsgIdentifier=516  MsgLength=8  SignalInfo=CumuTime_All$24$32$2$2$1$0$1.000000e-01$0$0$4294967295$#  NSignals=1  IDPort=off  TimestampPort=off  ErrorPort=off  RemotePort=off  LengthPort=off  StatusPort=off  StartBits=str2num('[int32(24)]')  SignalSizes=str2num('[int32(32)]')  ByteOrders=str2num('[int32(2)]')  DataTypes=str2num('[int32(2)]')  MultiplexTypes=str2num('[int32(1)]')  MultiplexValues=str2num('[double(0)]')  Factors=str2num('[double(1.000000e-01)]')  Offsets=str2num('[double(0)]')  Minimums=str2num('[double(0)]')  Maximums=str2num('[double(4294967295)]')  ApplyMinMax=off
      settings: SourceProductName=Simulink Real-Time  SourceProductBaseCode=XP  DataFormat=CANdb specified signals
  Constant1 : Constant  Value=0  OutDataTypeStr=uint8
  Constant4 : Constant  Value=0  OutDataTypeStr=uint8
  Constant5 : Constant  Value=0  OutDataTypeStr=uint8
  Data Type Conversion{,14..15,17} (4 alike) : DataTypeConversion  OutDataTypeStr=uint8
  Data Type Conversion18 : DataTypeConversion  OutDataTypeStr=uint32
  Data Type Conversion19 : DataTypeConversion  OutDataTypeStr=double
  Message : Outport
  wires:
  Constant4/1 -> Data Type Conversion15/1
  length/1 -> Data Type Conversion14/1
  data/1 -> Bus Creator/7  "Data"
  Data Type Conversion18/1 -> Bus Creator/5  "ID"
  Constant1/1 -> Data Type Conversion/1
  Constant5/1 -> Data Type Conversion17/1
  ID/1 -> Data Type Conversion18/1
  Data Type Conversion19/1 -> Bus Creator/6  "Timestamp"
  timestamp/1 -> Data Type Conversion19/1
  Data Type Conversion17/1 -> Bus Creator/4  "Error"
  Bus Creator/1 -> CAN Unpack6/1  "CAN_Msg_In"
  Data Type Conversion/1 -> Bus Creator/1  "Extended"
  Data Type Conversion14/1 -> Bus Creator/2  "Length"
  Data Type Conversion15/1 -> Bus Creator/3  "Remote"
  Bus Creator1/1 -> Message/1

== system ZT_VehCtrl_18B_CAN/SigIn/CAN0 /BMS HeatInfor/UNPACK ==
  ID : Inport
  data : Inport  Port=2
  length : Inport  Port=3
  timestamp : Inport  Port=4
  Action Port : ActionPort
  Bus Creator : BusCreator  Inputs=7  OutDataTypeStr=Bus: CAN_MESSAGE_BUS  NonVirtualBus=on
  Bus Creator1 : BusCreator  Inputs=2
  CAN Unpack6 : canmsglib/CAN Unpack  CANdbFile=D:\VCU\VCU_SL_ZhengZhou\ZT2\模型与接口\CAN_DBC\整车CANA_GBK.dbc  MsgList=(none)  MsgName=BMS_HeatInfor  MsgIDType=Standard (11-bit identifier)  MsgIdentifier=520  MsgLength=8  SignalInfo=BuzzerControl$40$16$2$2$1$0$1$0$0$1$#HeatCur$8$16$2$2$1$0$1.000000e-01$0$0$1000$#HeatCur$24$16$2$2$1$0$1.000000e-01$-1000$-1000$1000$#  NSignals=3  IDPort=off  TimestampPort=off  ErrorPort=off  RemotePort=off  LengthPort=off  StatusPort=off  StartBits=str2num('[int32(40);int32(8);int32(24)]')  SignalSizes=str2num('[int32(16);int32(16);int32(16)]')  ByteOrders=str2num('[int32(2);int32(2);int32(2)]')  DataTypes=str2num('[int32(2);int32(2);int32(2)]')  MultiplexTypes=str2num('[int32(1);int32(1);int32(1)]')  MultiplexValues=str2num('[double(0);double(0);double(0)]')  Factors=str2num('[double(1);double(1.000000e-01);double(1.000000e-01)]')  Offsets=str2num('[double(0);double(0);double(-1000)]')  Minimums=str2num('[double(0);double(0);double(-1000)]')  Maximums=str2num('[double(1);double(1000);double(1000)]')  ApplyMinMax=off
      settings: SourceProductName=Simulink Real-Time  SourceProductBaseCode=XP  DataFormat=CANdb specified signals
  Constant1 : Constant  Value=0  OutDataTypeStr=uint8
  Constant4 : Constant  Value=0  OutDataTypeStr=uint8
  Constant5 : Constant  Value=0  OutDataTypeStr=uint8
  Data Type Conversion{,14..15,17} (4 alike) : DataTypeConversion  OutDataTypeStr=uint8
  Data Type Conversion18 : DataTypeConversion  OutDataTypeStr=uint32
  Data Type Conversion19 : DataTypeConversion  OutDataTypeStr=double
  Message : Outport
  wires:
  Constant4/1 -> Data Type Conversion15/1
  length/1 -> Data Type Conversion14/1
  data/1 -> Bus Creator/7  "Data"
  Data Type Conversion18/1 -> Bus Creator/5  "ID"
  Constant1/1 -> Data Type Conversion/1
  Constant5/1 -> Data Type Conversion17/1
  ID/1 -> Data Type Conversion18/1
  Data Type Conversion19/1 -> Bus Creator/6  "Timestamp"
  timestamp/1 -> Data Type Conversion19/1
  Data Type Conversion17/1 -> Bus Creator/4  "Error"
  Bus Creator/1 -> CAN Unpack6/1  "CAN_Msg_In"
  Data Type Conversion/1 -> Bus Creator/1  "Extended"
  Data Type Conversion14/1 -> Bus Creator/2  "Length"
  Data Type Conversion15/1 -> Bus Creator/3  "Remote"
  Bus Creator1/1 -> Message/1

== system ZT_VehCtrl_18B_CAN/SigIn/CAN0 /BMS Power Infor/UNPACK ==
  ID : Inport
  data : Inport  Port=2
  length : Inport  Port=3
  timestamp : Inport  Port=4
  Action Port : ActionPort  ActionType=case
  Add : Sum
  Bus Creator : BusCreator  Inputs=7  OutDataTypeStr=Bus: CAN_MESSAGE_BUS  NonVirtualBus=on
  Bus Creator1 : BusCreator  Inputs=3
  CAN Unpack6 : canmsglib/CAN Unpack  CANdbFile=D:\VCU\VCU_SL_ZhengZhou\ZT2\模型与接口\CAN_DBC\整车CANA_GBK.dbc  MsgList=(none)  MsgName=BMS_Power_Infor  MsgIDType=Standard (11-bit identifier)  MsgIdentifier=529  MsgLength=8  SignalInfo=BMS_BatteryPower$40$16$2$2$1$0$1.000000e-02$-100$-100$100$#BMS_InsulationResistance$8$16$2$2$1$0$1$0$0$60$#BMS_RemainingChargingTime$24$16$2$2$1$0$1$0$0$1800$#  NSignals=3  IDPort=off  TimestampPort=off  ErrorPort=off  RemotePort=off  LengthPort=off  StatusPort=off  StartBits=str2num('[int32(40);int32(8);int32(24)]')  SignalSizes=str2num('[int32(16);int32(16);int32(16)]')  ByteOrders=str2num('[int32(2);int32(2);int32(2)]')  DataTypes=str2num('[int32(2);int32(2);int32(2)]')  MultiplexTypes=str2num('[int32(1);int32(1);int32(1)]')  MultiplexValues=str2num('[double(0);double(0);double(0)]')  Factors=str2num('[double(1.000000e-02);double(1);double(1)]')  Offsets=str2num('[double(-100);double(0);double(0)]')  Minimums=str2num('[double(-100);double(0);double(0)]')  Maximums=str2num('[double(100);double(60);double(1800)]')  ApplyMinMax=off
      settings: SourceProductName=Simulink Real-Time  SourceProductBaseCode=XP  DataFormat=CANdb specified signals
  Constant : Constant  OutDataTypeStr=uint8
  Constant1 : Constant  Value=0  OutDataTypeStr=uint8
  Constant4 : Constant  Value=0  OutDataTypeStr=uint8
  Constant5 : Constant  Value=0  OutDataTypeStr=uint8
  Data Store Read : DataStoreRead  DataStoreName=Cnt_BMS4
  Data Store Write : DataStoreWrite  DataStoreName=Cnt_BMS4
  Data Type Conversion{,14..15,17} (4 alike) : DataTypeConversion  OutDataTypeStr=uint8
  Data Type Conversion1 : DataTypeConversion  OutDataTypeStr=single
  Data Type Conversion18 : DataTypeConversion  OutDataTypeStr=uint32
  Data Type Conversion19 : DataTypeConversion  OutDataTypeStr=double
  Data Type Conversion2 : DataTypeConversion  OutDataTypeStr=single
  Data Type Conversion3 : DataTypeConversion  OutDataTypeStr=single
  Message : Outport
  wires:
  Constant4/1 -> Data Type Conversion15/1
  length/1 -> Data Type Conversion14/1
  data/1 -> Bus Creator/7  "Data"
  Data Type Conversion18/1 -> Bus Creator/5  "ID"
  Constant1/1 -> Data Type Conversion/1
  Constant5/1 -> Data Type Conversion17/1
  ID/1 -> Data Type Conversion18/1
  Data Type Conversion19/1 -> Bus Creator/6  "Timestamp"
  timestamp/1 -> Data Type Conversion19/1
  Data Type Conversion17/1 -> Bus Creator/4  "Error"
  Bus Creator/1 -> CAN Unpack6/1  "CAN_Msg_In"
  Data Type Conversion/1 -> Bus Creator/1  "Extended"
  Data Type Conversion14/1 -> Bus Creator/2  "Length"
  Data Type Conversion15/1 -> Bus Creator/3  "Remote"
  Bus Creator1/1 -> Message/1
  CAN Unpack6/1 -> Data Type Conversion3/1
  CAN Unpack6/2 -> Data Type Conversion2/1
  CAN Unpack6/3 -> Data Type Conversion1/1
  Data Type Conversion1/1 -> Bus Creator1/3  "BMS_RemainingChargingTime"
  Data Type Conversion2/1 -> Bus Creator1/2  "BMS_InsulationResistance"
  Data Type Conversion3/1 -> Bus Creator1/1  "BMS_BatteryPower"
  Add/1 -> Data Store Write/1
  Constant/1 -> Add/2
  Data Store Read/1 -> Add/1

== system ZT_VehCtrl_18B_CAN/SigIn/CAN0 /BMS StartDia_Infor1/UNPACK ==
  ID : Inport
  data : Inport  Port=2
  length : Inport  Port=3
  timestamp : Inport  Port=4
  Action Port : ActionPort
  Bus Creator : BusCreator  Inputs=7  OutDataTypeStr=Bus: CAN_MESSAGE_BUS  NonVirtualBus=on
  Bus Creator1 : BusCreator  Inputs=6
  CAN Unpack6 : canmsglib/CAN Unpack  CANdbFile=D:\VCU\VCU_SL_ZhengZhou\ZT2\模型与接口\CAN_DBC\整车CANA_GBK.dbc  MsgList=(none)  MsgName=BMS_StartDia_Infor1  MsgIDType=Standard (11-bit identifier)  MsgIdentifier=518  MsgLength=8  SignalInfo=Dchg_DiaFaultAction$32$8$2$2$1$0$1$0$0$255$#Dchg_DiaFaultFlag$24$8$2$2$1$0$1$0$0$255$#Dchg_DiaOtherFault$40$8$2$2$1$0$1$0$0$255$#Dchg_StartDiaFault$16$8$2$2$1$0$1$0$0$255$#SocStartDia_EmptyCalib$8$8$2$2$1$0$1$0$0$255$#SocStartDia_FullCalib$0$8$2$2$1$0$1$0$0$255$#  NSignals=6  IDPort=off  TimestampPort=off  ErrorPort=off  RemotePort=off  LengthPort=off  StatusPort=off  StartBits=str2num('[int32(32);int32(24);int32(40);int32(16);int32(8);int32(0)]')  SignalSizes=str2num('[int32(8);int32(8);int32(8);int32(8);int32(8);int32(8)]')  ByteOrders=str2num('[int32(2);int32(2);int32(2);int32(2);int32(2);int32(2)]')  DataTypes=str2num('[int32(2);int32(2);int32(2);int32(2);int32(2);int32(2)]')  MultiplexTypes=str2num('[int32(1);int32(1);int32(1);int32(1);int32(1);int32(1)]')  MultiplexValues=str2num('[double(0);double(0);double(0);double(0);double(0);double(0)]')  Factors=str2num('[double(1);double(1);double(1);double(1);double(1);double(1)]')  Offsets=str2num('[double(0);double(0);double(0);double(0);double(0);double(0)]')  Minimums=str2num('[double(0);double(0);double(0);double(0);double(0);double(0)]')  Maximums=str2num('[double(255);double(255);double(255);double(255);double(255);double(255)]')  ApplyMinMax=off
      settings: SourceProductName=Simulink Real-Time  SourceProductBaseCode=XP  DataFormat=CANdb specified signals
  Constant1 : Constant  Value=0  OutDataTypeStr=uint8
  Constant4 : Constant  Value=0  OutDataTypeStr=uint8
  Constant5 : Constant  Value=0  OutDataTypeStr=uint8
  Data Type Conversion{,14..15,17} (4 alike) : DataTypeConversion  OutDataTypeStr=uint8
  Data Type Conversion1 : DataTypeConversion
  Data Type Conversion18 : DataTypeConversion  OutDataTypeStr=uint32
  Data Type Conversion19 : DataTypeConversion  OutDataTypeStr=double
  Message : Outport
  wires:
  Constant4/1 -> Data Type Conversion15/1
  length/1 -> Data Type Conversion14/1
  data/1 -> Bus Creator/7  "Data"
  Data Type Conversion18/1 -> Bus Creator/5  "ID"
  Constant1/1 -> Data Type Conversion/1
  Constant5/1 -> Data Type Conversion17/1
  ID/1 -> Data Type Conversion18/1
  Data Type Conversion19/1 -> Bus Creator/6  "Timestamp"
  timestamp/1 -> Data Type Conversion19/1
  Data Type Conversion17/1 -> Bus Creator/4  "Error"
  Bus Creator/1 -> CAN Unpack6/1  "CAN_Msg_In"
  Data Type Conversion/1 -> Bus Creator/1  "Extended"
  Data Type Conversion14/1 -> Bus Creator/2  "Length"
  Data Type Conversion15/1 -> Bus Creator/3  "Remote"
  Bus Creator1/1 -> Message/1
  CAN Unpack6/6 -> Data Type Conversion1/1
  CAN Unpack6/5 -> Bus Creator1/5
  CAN Unpack6/4 -> Bus Creator1/4
  CAN Unpack6/3 -> Bus Creator1/3
  CAN Unpack6/2 -> Bus Creator1/2
  CAN Unpack6/1 -> Bus Creator1/1
  Data Type Conversion1/1 -> Bus Creator1/6

== system ZT_VehCtrl_18B_CAN/SigIn/CAN0 /BMS StartDia_Infor2/UNPACK ==
  ID : Inport
  data : Inport  Port=2
  length : Inport  Port=3
  timestamp : Inport  Port=4
  Action Port : ActionPort
  Bus Creator : BusCreator  Inputs=7  OutDataTypeStr=Bus: CAN_MESSAGE_BUS  NonVirtualBus=on
  Bus Creator1 : BusCreator  Inputs=2
  CAN Unpack6 : canmsglib/CAN Unpack  CANdbFile=D:\VCU\VCU_SL_ZhengZhou\ZT2\模型与接口\CAN_DBC\整车CANA_GBK.dbc  MsgList=(none)  MsgName=BMS_StartDia_Infor2  MsgIDType=Standard (11-bit identifier)  MsgIdentifier=519  MsgLength=8  SignalInfo=Chg_DiaFaultAction$16$8$2$2$1$0$1$0$0$255$#Chg_DiaFaultFlag$8$8$2$2$1$0$1$0$0$255$#Chg_DiaOtherFault$24$8$2$2$1$0$1$0$0$255$#Chg_StartDiaFault$0$8$2$2$1$0$1$0$0$255$#OBC_FaultCode$40$16$2$2$1$0$1$0$0$255$#  NSignals=5  IDPort=off  TimestampPort=off  ErrorPort=off  RemotePort=off  LengthPort=off  StatusPort=off  StartBits=str2num('[int32(16);int32(8);int32(24);int32(0);int32(40)]')  SignalSizes=str2num('[int32(8);int32(8);int32(8);int32(8);int32(16)]')  ByteOrders=str2num('[int32(2);int32(2);int32(2);int32(2);int32(2)]')  DataTypes=str2num('[int32(2);int32(2);int32(2);int32(2);int32(2)]')  MultiplexTypes=str2num('[int32(1);int32(1);int32(1);int32(1);int32(1)]')  MultiplexValues=str2num('[double(0);double(0);double(0);double(0);double(0)]')  Factors=str2num('[double(1);double(1);double(1);double(1);double(1)]')  Offsets=str2num('[double(0);double(0);double(0);double(0);double(0)]')  Minimums=str2num('[double(0);double(0);double(0);double(0);double(0)]')  Maximums=str2num('[double(255);double(255);double(255);double(255);double(255)]')  ApplyMinMax=off
      settings: SourceProductName=Simulink Real-Time  SourceProductBaseCode=XP  DataFormat=CANdb specified signals
  Constant1 : Constant  Value=0  OutDataTypeStr=uint8
  Constant4 : Constant  Value=0  OutDataTypeStr=uint8
  Constant5 : Constant  Value=0  OutDataTypeStr=uint8
  Data Type Conversion{,14..15,17} (4 alike) : DataTypeConversion  OutDataTypeStr=uint8
  Data Type Conversion18 : DataTypeConversion  OutDataTypeStr=uint32
  Data Type Conversion19 : DataTypeConversion  OutDataTypeStr=double
  Message : Outport
  wires:
  Bus Creator1/1 -> Message/1
  Data Type Conversion15/1 -> Bus Creator/3  "Remote"
  Data Type Conversion14/1 -> Bus Creator/2  "Length"
  Data Type Conversion/1 -> Bus Creator/1  "Extended"
  Bus Creator/1 -> CAN Unpack6/1  "CAN_Msg_In"
  Data Type Conversion17/1 -> Bus Creator/4  "Error"
  timestamp/1 -> Data Type Conversion19/1
  Data Type Conversion19/1 -> Bus Creator/6  "Timestamp"
  ID/1 -> Data Type Conversion18/1
  Constant5/1 -> Data Type Conversion17/1
  Constant1/1 -> Data Type Conversion/1
  Data Type Conversion18/1 -> Bus Creator/5  "ID"
  data/1 -> Bus Creator/7  "Data"
  length/1 -> Data Type Conversion14/1
  Constant4/1 -> Data Type Conversion15/1
